simulink model "ADCSSimulator"  (R2024a)
settings: Solver=ode4  StartTime=0.0  StopTime=600  FixedStep=0.01  MaxStep=0.1  RelTol=1e-3  AbsTol=1e-3
values from neighbouring files (symbols this model uses):
  ActuatorAllocationMatrix = ActuatorPhysicalMatrix' * inv(ActuatorPhysicalMatrix * ActuatorPhysicalMatrix')    [set_Init.m]
  ActuatorPhysicalMatrix = [1, 0, 0, 0 ... (first row only)    [set_Init.m]
  albedo_irradiance = 300    [set_Init.m]
  b = 0    [set_Init.m]
  Cd = 2.2    [set_Init.m]
  h_bias = [0; 0; 0]    [set_Init.m]
  J = 4.0e-3 / 628    (= 6.36942675159e-06)    [set_Init.m]
  k_Bdot = ((4 * pi * 0.5236 * 0.0055) / (5677.2 * (4.5e-5)^2))    (= 3147.8423197)    [set_Init.m]
  K_E = K_T    (= 0.0022)    [set_Init.m]
  K_T = 0.0022    [set_Init.m]
  P0 = blkdiag(P0_att, P0_bias)    [set_Init.m]
  P0_att = eye(3) * initial_variance_rad2    [set_Init.m]
  PowerVoltageBus_01 = 3.3    [set_Init.m]
  PowerVoltageBus_02 = 3.3    [set_Init.m]
  PowerVoltageBus_03 = 3.3    [set_Init.m]
  PowerVoltageBus_04 = 3.3    [set_Init.m]
  PowerVoltageBus_05 = 3.3    [set_Init.m]
  PowerVoltageBus_06 = 3.3    [set_Init.m]
  PowerVoltageBus_07 = 3.3    [set_Init.m]
  PowerVoltageBus_08 = 3.3    [set_Init.m]
  PowerVoltageBus_09 = 3.3    [set_Init.m]
  PowerVoltageBus_10 = 3.3    [set_Init.m]
  PowerVoltageBus_11 = 3.3    [set_Init.m]
  PowerVoltageBus_12 = 0.0    (= 0)    [set_Init.m]
  PowerVoltageBus_13 = 0.0    (= 0)    [set_Init.m]
  PowerVoltageBus_14 = 0.0    (= 0)    [set_Init.m]
  PowerVoltageBus_15 = 0.0    (= 0)    [set_Init.m]
  R = 2.0    (= 2)    [set_Init.m]
  ressidual_m = [3e-4; -2e-4; 1e-4]    [set_Init.m]
  solar_irradiance = 1361    [set_Init.m]
  surface_areas = [A_xy, A_yz, A_xz, A_xy, A_yz, A_xz]    [set_Init.m]
  surface_normals_body = [eye(3) -eye(3)]    [set_Init.m]
  surface_positions_body = [       hx,   0,   0 ... (first row only)    [set_Init.m]
  surface_reflectivities = [0.9 0.8 0.9 0.9 0.9 0.9]    [set_Init.m]
  Switch_01 = 1    [set_Init.m]
  Switch_02 = 1    [set_Init.m]
  Switch_03 = 1    [set_Init.m]
  Switch_04 = 1    [set_Init.m]
  Switch_05 = 1    [set_Init.m]
  Switch_06 = 1    [set_Init.m]
  Switch_07 = 1    [set_Init.m]
  Switch_08 = 1    [set_Init.m]
  Switch_09 = 1    [set_Init.m]
  Switch_10 = 1    [set_Init.m]
  Switch_11 = 1    [set_Init.m]
  Switch_12 = 0    [set_Init.m]
  Switch_13 = 0    [set_Init.m]
  Switch_14 = 0    [set_Init.m]
  Switch_15 = 0    [set_Init.m]
  visSampleTime = 0.1    [set_Init.m]
undefined symbols (not defined in the file or in its folder): attitude, Controller, epoch, IAU, juliandate, Kd, km, Kp, m, rad, s, satellite, SGP4_parameters, simulator, UKF_parameters, WMM2020
libraries: sharedtransform x27, aerolibutil x22, aerolibconvert2 x18, simulink_extras x16, matrix_library x6, aerolibtransform2 x4, vrlib x2, aerolibgravity2 x2, aerolibobsolete x1, aerolibattitudesys x1, simulink x1
(part 2 of 8)

== system ADCSSimulator/ADCS/ADCS Software/Onboard Models ==
  Onboard Calendar : Inport
  Satellite Ephemeris [ICRF] : Inport  Port=2
  Transformers : Inport  Port=3
  Bus Creator : BusCreator  Inputs=2
  Bus Selector : BusSelector  OutputSignals=Satellite Position [ICRF] (m)
  Calendar1 : InportShadow
  Onboard Sun Ephemeris Calculator : Subsystem
  WMM : Subsystem
  Onboard Models : Outport
  wires:
  Calendar1/1 -> WMM/2(Calendar)
  WMM/1(Onboard Magnetic Field (T)) -> Bus Creator/2  "Onboard Magnetic Field"
  Onboard Sun Ephemeris Calculator/1(Onboard Sun Ephemeris [ICRF]) -> Bus Creator/1  "Onboard Sun Ephemeris"
  Transformers/1 -> WMM/3(Transformers)
  Satellite Ephemeris [ICRF]/1 -> Bus Selector/1
  Onboard Calendar/1 -> Onboard Sun Ephemeris Calculator/1(Onboard Calendar)
  Bus Selector/1 -> WMM/1(Satellite Position [ICRF] (m))  "<Satellite Position [ICRF] (m)>"
  Bus Creator/1 -> Onboard Models/1

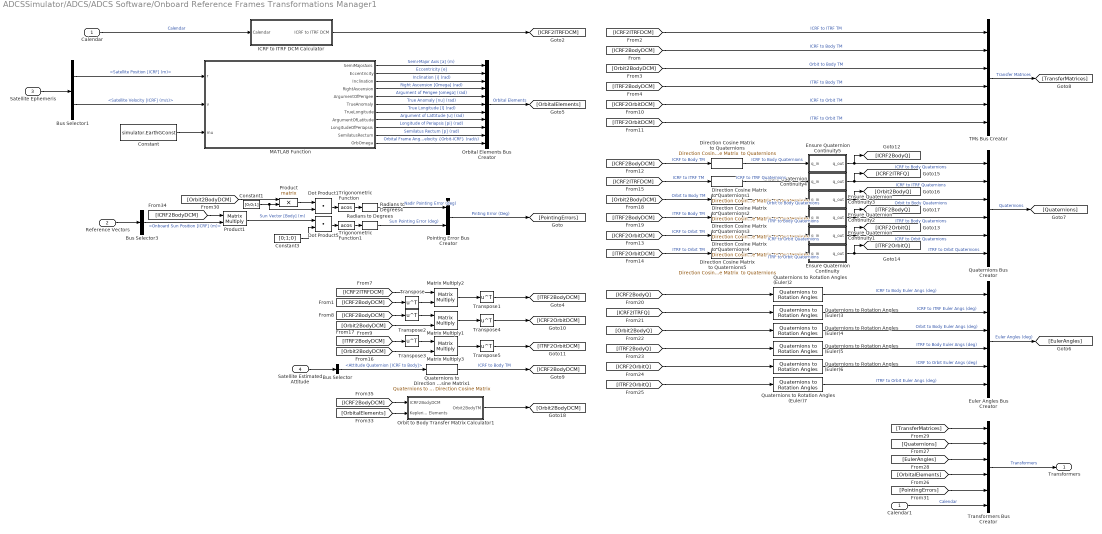
== system ADCSSimulator/ADCS/ADCS Software/Onboard Reference Frames Transformations Manager1 ==
  Calendar : Inport
  Reference Vectors : Inport  Port=2
  Satellite Ephemeris : Inport  Port=3
  Satellite Estimated Attitude : Inport  Port=4
  Bus Selector : BusSelector  OutputSignals=Attitude Quaternion [ICRF to Body]
  Bus Selector1 : BusSelector  OutputSignals=Satellite Position [ICRF] (m),Satellite Velocity [ICRF] (m/s)
  Bus Selector3 : BusSelector  OutputSignals=Onboard Sun Ephemeris.Onboard Sun Position [ICRF] (m)
  Calendar1 : InportShadow
  Constant : Constant  Value=simulator.EarthGConst
  Constant1 : Constant  Value=[0;0;1]
  Constant3 : Constant  Value=[0;1;0]
  Direction Cosine Matrix to Quaternions{,1..5} (6 alike) : sharedtransform/Direction Cosine Matrix  to Quaternions  aMode=0  action=None  tolerance=eps(2)
  Dot Product1 : DotProduct  OutDataTypeStr=Inherit: Inherit via internal rule
  Dot Product5 : DotProduct  OutDataTypeStr=Inherit: Inherit via internal rule
  Ensure Quaternion Continuity : Subsystem
  Ensure Quaternion Continuity1 : Subsystem
  Ensure Quaternion Continuity2 : Subsystem
  Ensure Quaternion Continuity3 : Subsystem
  Ensure Quaternion Continuity4 : Subsystem
  Ensure Quaternion Continuity5 : Subsystem
  Euler Angles Bus Creator : BusCreator  Inputs=6
  ICRF to ITRF DCM Calculator : Subsystem
  MATLAB Function : MATLAB Function  TreatAsAtomicUnit=on
  Matrix Multiply1 : Product  Multiplication=Matrix(*)
  Matrix Multiply2 : Product  Multiplication=Matrix(*)
  Matrix Multiply3 : Product  Multiplication=Matrix(*)
  Orbit to Body Transfer Matrix Calculator1 : Subsystem
  Orbital Elements Bus Creator : BusCreator  Inputs=11
  Pointing Error Bus Creator : BusCreator  Inputs=2
  Product : Product  Multiplication=Matrix(*)
  Product1 : Product  Multiplication=Matrix(*)
  Quaternions Bus Creator : BusCreator  Inputs=6
  Quaternions to Direction Cosine Matrix1 : sharedtransform/Quaternions to  Direction Cosine Matrix  aMode=aMode
  Quaternions to Rotation Angles (Euler){2..7} (6 alike) : sharedtransform/Quaternions to Rotation Angles  rotationOrder=XYZ  aMode=aMode
  Radians to Degrees : simulink_extras/Transformations/Radians to Degrees
  Radians to Degrees4 : simulink_extras/Transformations/Radians to Degrees
  TMs Bus Creator : BusCreator  Inputs=6
  Transformers Bus Creator : BusCreator  Inputs=6
  Transpose{,1..5} (6 alike) : Math  Operator=transpose
  Trigonometric Function : Trigonometry  Operator=acos
  Trigonometric Function1 : Trigonometry  Operator=acos  OutputSignalType=real
  Transformers : Outport
  wires:
  MATLAB Function/7(TrueLongitude) -> Orbital Elements Bus Creator/7  "True Longitude [l] (rad)"
  Ensure Quaternion Continuity3/1(q_out) -> Quaternions Bus Creator/3, [Orbit2BodyQ]  "Orbit to Body Quaternions"
  [Orbit2BodyQ] -> Quaternions to Rotation Angles (Euler)4/1
  [ITRF2OrbitQ] -> Quaternions to Rotation Angles (Euler)7/1
  [ITRF2OrbitDCM] -> Direction Cosine Matrix to Quaternions5/1  "ITRF to Orbit TM"
  Bus Selector1/2 -> MATLAB Function/2(v)  "<Satellite Velocity [ICRF] (m/s)>"
  [ICRF2ITRFQ] -> Quaternions to Rotation Angles (Euler)3/1
  [ICRF2OrbitQ] -> Quaternions to Rotation Angles (Euler)6/1
  [ICRF2BodyDCM] -> Transpose2/1
  [EulerAngles] -> Transformers Bus Creator/3
  MATLAB Function/6(TrueAnomaly) -> Orbital Elements Bus Creator/6  "True Anomaly [nu] (rad)"
  MATLAB Function/5(ArgumentOfPerigee) -> Orbital Elements Bus Creator/5  "Argument of Perigee [omega] (rad)"
  Transformers Bus Creator/1 -> Transformers/1  "Transformers"
  MATLAB Function/4(RightAscension) -> Orbital Elements Bus Creator/4  "Right Ascension [Omega] (rad)"
  MATLAB Function/10(SemilatusRectum) -> Orbital Elements Bus Creator/10  "Semilatus Rectum [p] (rad)"
  MATLAB Function/9(LongitudeOfPeriapsis) -> Orbital Elements Bus Creator/9  "Longitude of Periapsis [pi] (rad)"
  Ensure Quaternion Continuity1/1(q_out) -> Quaternions Bus Creator/5, [ICRF2OrbitQ]  "ICRF to Orbit Quaternions"
  MATLAB Function/8(ArgumentOfLatitude) -> Orbital Elements Bus Creator/8  "Argument of Lattitude [u] (rad)"
  MATLAB Function/1(SemiMajorAxis) -> Orbital Elements Bus Creator/1  "Semi-Major Axis [a] (m)"
  Reference Vectors/1 -> Bus Selector3/1
  Dot Product5/1 -> Trigonometric Function1/1
  [ICRF2BodyDCM] -> Transpose/1
  Matrix Multiply2/1 -> Transpose1/1
  Bus Selector1/1 -> MATLAB Function/1(r)  "<Satellite Position [ICRF] (m)>"
  [Orbit2BodyDCM] -> Matrix Multiply1/2
  Orbital Elements Bus Creator/1 -> [OrbitalElements]  "Orbital Elements"
  Transpose1/1 -> [ITRF2BodyDCM]
  Trigonometric Function/1 -> Radians to Degrees4/1
  Matrix Multiply3/1 -> Transpose5/1
  Constant3/1 -> Dot Product5/2
  [OrbitalElements] -> Transformers Bus Creator/4
  [ITRF2BodyDCM] -> Transpose3/1
  [Orbit2BodyDCM] -> Matrix Multiply3/2
  Radians to Degrees4/1 -> Pointing Error Bus Creator/1  "Nadir Pointing Error (deg)"
  Radians to Degrees/1 -> Pointing Error Bus Creator/2  "Sun Pointing Error (deg)"
  Calendar/1 -> ICRF to ITRF DCM Calculator/1(Calendar)  "Calendar"
  Pointing Error Bus Creator/1 -> [PointingErrors]  "Pinting Error (Deg)"
  MATLAB Function/11(OrbOmega) -> Orbital Elements Bus Creator/11  "Orbital Frame Angular Velocity {Orbit-ICRF} (rad/s)"
  Constant/1 -> MATLAB Function/3(mu)
  [Orbit2BodyDCM] -> Direction Cosine Matrix to Quaternions2/1  "Orbit to Body TM"
  [ICRF2ITRFDCM] -> TMs Bus Creator/1  "ICRF to ITRF TM"
  [ICRF2BodyDCM] -> TMs Bus Creator/2  "ICRF to Body TM"
  [PointingErrors] -> Transformers Bus Creator/5
  Transpose/1 -> Matrix Multiply2/2
  [Orbit2BodyDCM] -> Product/1
  Direction Cosine Matrix to Quaternions/1 -> Ensure Quaternion Continuity5/1(q_in)  "ICRF to Body Quaternions"
  [ICRF2OrbitDCM] -> TMs Bus Creator/5  "ICRF to Orbit TM"
  Ensure Quaternion Continuity/1(q_out) -> Quaternions Bus Creator/6, [ITRF2OrbitQ]  "ITRF to Orbit Quaternions"
  Direction Cosine Matrix to Quaternions3/1 -> Ensure Quaternion Continuity2/1(q_in)  "ITRF to Body Quaternions"
  [ICRF2BodyQ] -> Quaternions to Rotation Angles (Euler)2/1
  Constant1/1 -> Product/2, Dot Product1/2
  [ITRF2BodyDCM] -> TMs Bus Creator/4  "ITRF to Body TM"
  Quaternions to Rotation Angles (Euler)7/1 -> Euler Angles Bus Creator/6  "ITRF to Orbit Euler Angs (deg)"
  [Quaternions] -> Transformers Bus Creator/2
  [ITRF2OrbitDCM] -> TMs Bus Creator/6  "ITRF to Orbit TM"
  [ICRF2ITRFDCM] -> Matrix Multiply2/1
  Bus Selector/1 -> Quaternions to Direction Cosine Matrix1/1  "<Attitude Quaternion [ICRF to Body]>"
  Calendar1/1 -> Transformers Bus Creator/6  "Calendar"
  MATLAB Function/2(Eccentricity) -> Orbital Elements Bus Creator/2  "Eccentricity [e]"
  Ensure Quaternion Continuity4/1(q_out) -> Quaternions Bus Creator/2, [ICRF2ITRFQ]  "ICRF to ITRF Quaternions"
  Satellite Ephemeris/1 -> Bus Selector1/1
  Quaternions Bus Creator/1 -> [Quaternions]  "Quaternions"
  [ICRF2ITRFDCM] -> Direction Cosine Matrix to Quaternions1/1  "ICRF to ITRF TM"
  Matrix Multiply1/1 -> Transpose4/1
  Direction Cosine Matrix to Quaternions5/1 -> Ensure Quaternion Continuity/1(q_in)  "ITRF to Orbit Quaternions"
  Direction Cosine Matrix to Quaternions4/1 -> Ensure Quaternion Continuity1/1(q_in)  "ICRF to Orbit Quaternions"
  TMs Bus Creator/1 -> [TransferMatrices]  "Transfer Matrices"
  [ITRF2BodyDCM] -> Direction Cosine Matrix to Quaternions3/1  "ITRF to Body TM"
  Product1/1 -> Dot Product5/1  "Sun Vector [Body] (m)"
  Product/1 -> Dot Product1/1
  Ensure Quaternion Continuity2/1(q_out) -> Quaternions Bus Creator/4, [ITRF2BodyQ]  "ITRF to Body Quaternions"
  Direction Cosine Matrix to Quaternions2/1 -> Ensure Quaternion Continuity3/1(q_in)  "Orbit to Body Quaternions"
  Ensure Quaternion Continuity5/1(q_out) -> Quaternions Bus Creator/1, [ICRF2BodyQ]  "ICRF to Body Quaternions"
  Quaternions to Rotation Angles (Euler)5/1 -> Euler Angles Bus Creator/4  "ITRF to Body Euler Angs (deg)"
  Dot Product1/1 -> Trigonometric Function/1
  Direction Cosine Matrix to Quaternions1/1 -> Ensure Quaternion Continuity4/1(q_in)  "ICRF to ITRF Quaternions"
  Quaternions to Rotation Angles (Euler)2/1 -> Euler Angles Bus Creator/1  "ICRF to Body Euler Angs (deg)"
  Quaternions to Rotation Angles (Euler)3/1 -> Euler Angles Bus Creator/2  "ICRF to ITRF Euler Angs (deg)"
  Euler Angles Bus Creator/1 -> [EulerAngles]  "Euler Angles (deg)"
  MATLAB Function/3(Inclination) -> Orbital Elements Bus Creator/3  "Inclination [i] (rad)"
  [TransferMatrices] -> Transformers Bus Creator/1
  [ICRF2OrbitDCM] -> Direction Cosine Matrix to Quaternions4/1  "ICRF to Orbit TM"
  Quaternions to Rotation Angles (Euler)6/1 -> Euler Angles Bus Creator/5  "ICRF to Orbit Euler Angs (deg)"
  [ITRF2BodyQ] -> Quaternions to Rotation Angles (Euler)5/1
  [Orbit2BodyDCM] -> TMs Bus Creator/3  "Orbit to Body TM"
  Trigonometric Function1/1 -> Radians to Degrees/1
  Quaternions to Rotation Angles (Euler)4/1 -> Euler Angles Bus Creator/3  "Orbit to Body Euler Angs (deg)"
  [ICRF2BodyDCM] -> Direction Cosine Matrix to Quaternions/1  "ICRF to Body TM"
  [ICRF2BodyDCM] -> Product1/1
  Bus Selector3/1 -> Product1/2  "<Onboard Sun Position [ICRF] (m)>"
  ICRF to ITRF DCM Calculator/1(ICRF to ITRF DCM) -> [ICRF2ITRFDCM]
  Transpose2/1 -> Matrix Multiply1/1
  Transpose4/1 -> [ICRF2OrbitDCM]
  Transpose3/1 -> Matrix Multiply3/1
  Transpose5/1 -> [ITRF2OrbitDCM]
  [OrbitalElements] -> Orbit to Body Transfer Matrix Calculator1/2(Keplerian Elements)
  [ICRF2BodyDCM] -> Orbit to Body Transfer Matrix Calculator1/1(ICRF2BodyDCM)
  Quaternions to Direction Cosine Matrix1/1 -> [ICRF2BodyDCM]  "ICRF to Body TM"
  Orbit to Body Transfer Matrix Calculator1/1(Orbit2BodyTM) -> [Orbit2BodyDCM]
  Satellite Estimated Attitude/1 -> Bus Selector/1

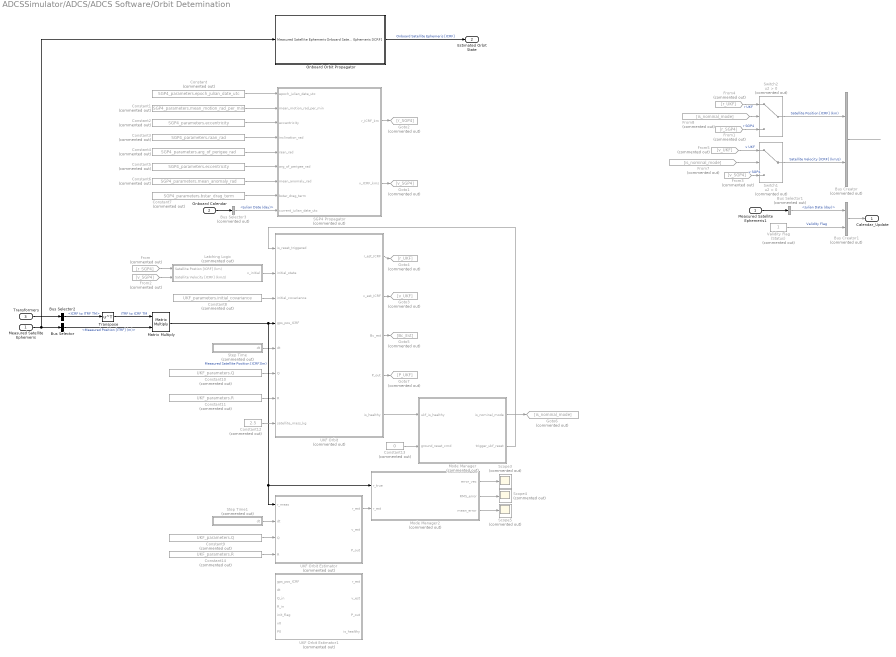
== system ADCSSimulator/ADCS/ADCS Software/Orbit Detemination ==
  Measured Satellite Ephemeris : Inport
  Onboard Calendar : Inport  Port=2
  Transformers : Inport  Port=3
  Bus Creator : BusCreator  Commented=on  Inputs=2
  Bus Creator1 : BusCreator  Commented=on  Inputs=2
  Bus Selector : BusSelector  OutputSignals=Measured Position [ITRF] (m)
  Bus Selector1 : BusSelector  Commented=on  OutputSignals=Julian Date (day)
  Bus Selector2 : BusSelector  OutputSignals=Transfer Matrices.ICRF to ITRF TM
  Bus Selector3 : BusSelector  Commented=on  OutputSignals=Julian Date (day)
  Constant : Constant  Commented=on  Value=SGP4_parameters.epoch_julian_date_utc
  Constant1 : Constant  Commented=on  Value=SGP4_parameters.mean_motion_rad_per_min
  Constant10 : Constant  Commented=on  Value=UKF_parameters.Q
  Constant11 : Constant  Commented=on  Value=UKF_parameters.R
  Constant12 : Constant  Commented=on  Value=2.5
  Constant13 : Constant  Commented=on  Value=0
  Constant14 : Constant  Commented=on  Value=UKF_parameters.R
  Constant2 : Constant  Commented=on  Value=SGP4_parameters.eccentricity
  Constant3 : Constant  Commented=on  Value=SGP4_parameters.raan_rad
  Constant4 : Constant  Commented=on  Value=SGP4_parameters.arg_of_perigee_rad
  Constant5 : Constant  Commented=on  Value=SGP4_parameters.eccentricity
  Constant6 : Constant  Commented=on  Value=SGP4_parameters.mean_anomaly_rad
  Constant7 : Constant  Commented=on  Value=SGP4_parameters.bstar_drag_term
  Constant8 : Constant  Commented=on  Value=UKF_parameters.initial_covariance
  Constant9 : Constant  Commented=on  Value=UKF_parameters.Q
  From : From  Commented=on  GotoTag=r_SGP4
  From1 : From  Commented=on  GotoTag=r_SGP4
  From2 : From  Commented=on  GotoTag=v_SGP4
  From3 : From  Commented=on  GotoTag=v_SGP4
  From4 : From  Commented=on  GotoTag=r_UKF
  From5 : From  Commented=on  GotoTag=v_UKF
  From7 : From  Commented=on  GotoTag=is_nominal_mode
  From8 : From  Commented=on  GotoTag=is_nominal_mode
  Goto1 : Goto  Commented=on  GotoTag=v_SGP4
  Goto2 : Goto  Commented=on  GotoTag=r_SGP4
  Goto3 : Goto  Commented=on  GotoTag=v_UKF
  Goto4 : Goto  Commented=on  GotoTag=r_UKF
  Goto5 : Goto  Commented=on  GotoTag=Bc_Est
  Goto6 : Goto  Commented=on  GotoTag=is_nominal_mode
  Goto7 : Goto  Commented=on  GotoTag=P_UKF
  Latching Logic : Subsystem  Commented=on
  Matrix Multiply : Product  Multiplication=Matrix(*)
  Measured Satellite Ephemeris1 : InportShadow
  Mode Manager : MATLAB Function  Commented=on  TreatAsAtomicUnit=on
  Mode Manager2 : MATLAB Function  Commented=on  TreatAsAtomicUnit=on
  "Onboard Orbit Propagator " : Subsystem
  SGP4 Propagator : MATLAB Function  Commented=on  TreatAsAtomicUnit=on
  Scope3 : Scope  Commented=on
  Scope4 : Scope  Commented=on
  Scope5 : Scope  Commented=on
  Step Time : Subsystem  Commented=on
  Step Time1 : Subsystem  Commented=on
  Switch1 : Switch  Commented=on  Criteria=u2 > Threshold  SaturateOnIntegerOverflow=off  InputSameDT=off
  Switch2 : Switch  Commented=on  Criteria=u2 > Threshold  SaturateOnIntegerOverflow=off  InputSameDT=off
  Transpose : Math  Operator=transpose
  "UKF Orbit " : MATLAB Function  Commented=on  TreatAsAtomicUnit=on  SystemSampleTime=1
  UKF Orbit Estimator : MATLAB Function  Commented=on  TreatAsAtomicUnit=on
  UKF Orbit Estimator1 : MATLAB Function  Commented=on  TreatAsAtomicUnit=on
  Validity Flag (Status) : Constant  Commented=on
  Calendar_Update : Outport
  Estimated Orbit State : Outport  Port=2
  wires:
  Constant/1 -> SGP4 Propagator/1(epoch_julian_date_utc)
  Constant1/1 -> SGP4 Propagator/2(mean_motion_rad_per_min)
  Constant2/1 -> SGP4 Propagator/3(eccentricity)
  Constant4/1 -> SGP4 Propagator/5(raan_rad)
  Constant5/1 -> SGP4 Propagator/6(arg_of_perigee_rad)
  Constant3/1 -> SGP4 Propagator/4(inclination_rad)
  Bus Selector/1 -> Matrix Multiply/2  "<Measured Position [ITRF] (m)>"
  Step Time/1(dt) -> "UKF Orbit "/5(dt)
  Constant8/1 -> "UKF Orbit "/3(initial_covariance)
  Constant10/1 -> "UKF Orbit "/6(Q)
  Constant11/1 -> "UKF Orbit "/7(R)
  Latching Logic/1(x_initial) -> "UKF Orbit "/2(initial_state)
  SGP4 Propagator/2(v_ICRF_kms) -> Goto1/1
  SGP4 Propagator/1(r_ICRF_km) -> Goto2/1
  From/1 -> Latching Logic/1(Satellite Postion [ICRF] (km))
  From2/1 -> Latching Logic/2(Satellite Velocity [ICRF] (km/s))
  "UKF Orbit "/3(Bc_est) -> Goto5/1
  Bus Creator/1 -> ?
  "UKF Orbit "/2(v_est_ICRF) -> Goto3/1
  "UKF Orbit "/1(r_est_ICRF) -> Goto4/1
  Switch2/1 -> Bus Creator/1  "Satellite Position [ICRF] (km)"
  Switch1/1 -> Bus Creator/2  "Satellite Velocity [ICRF] (km/s)"
  Constant6/1 -> SGP4 Propagator/7(mean_anomaly_rad)
  Measured Satellite Ephemeris1/1 -> Bus Selector1/1
  Bus Selector1/1 -> Bus Creator1/1  "<Julian Date (day)>"
  Validity Flag (Status)/1 -> Bus Creator1/2  "Validity Flag"
  Bus Creator1/1 -> Calendar_Update/1
  Bus Selector2/1 -> Transpose/1  "<ICRF to ITRF TM>"
  Transformers/1 -> Bus Selector2/1
  Transpose/1 -> Matrix Multiply/1  "ITRF to ICRF TM"
  Matrix Multiply/1 -> "UKF Orbit "/4(gps_pos_ICRF), UKF Orbit Estimator/1(r_meas), Mode Manager2/1(r_true)  "Measured Satellite Position [ICRF](m)"
  Onboard Calendar/1 -> Bus Selector3/1
  Bus Selector3/1 -> SGP4 Propagator/9(current_julian_date_utc)  "<Julian Date (day)>"
  Constant12/1 -> "UKF Orbit "/8(satellite_mass_kg)
  Mode Manager/2(trigger_ukf_reset) -> "UKF Orbit "/1(is_reset_triggered)
  "UKF Orbit "/5(is_healthy) -> Mode Manager/1(ukf_is_healthy)
  From1/1 -> Switch2/3  "r SGP4"
  From4/1 -> Switch2/1  "r UKF"
  Constant13/1 -> Mode Manager/2(ground_reset_cmd)
  Mode Manager/1(is_nominal_mode) -> Goto6/1
  From8/1 -> Switch2/2
  From7/1 -> Switch1/2
  From3/1 -> Switch1/3  "v SGP4"
  From5/1 -> Switch1/1  "v UKF"
  "UKF Orbit "/4(P_out) -> Goto7/1
  Constant7/1 -> SGP4 Propagator/8(bstar_drag_term)
  "Onboard Orbit Propagator "/1(Onboard Satellite Ephemeris [ICRF]) -> Estimated Orbit State/1  "Onboard Satellite Ephemeris [ICRF]"
  Measured Satellite Ephemeris/1 -> "Onboard Orbit Propagator "/1(Measured Satellite Ephemeris), Bus Selector/1
  Constant14/1 -> UKF Orbit Estimator/4(R)
  Step Time1/1(dt) -> UKF Orbit Estimator/2(dt)
  Constant9/1 -> UKF Orbit Estimator/3(Q)
  UKF Orbit Estimator/1(r_est) -> Mode Manager2/2(r_est)
  Mode Manager2/1(error_vec) -> Scope3/1
  Mode Manager2/2(RMS_error) -> Scope4/1
  Mode Manager2/3(mean_error) -> Scope5/1

== system ADCSSimulator/ADCS/Environment Model/Attitude Dynamics & Kynematics ==
  Transformers : Inport
  Actuators : Inport  Port=2
  Disturbances : Inport  Port=3
  Bus Selector : BusSelector  OutputSignals=Transfer Matrices.Orbit to Body TM,Orbital Elements.Orbital Frame Angular Velocity {Orbit-ICRF} (rad/s)
  Bus Selector1 : BusSelector  OutputSignals=RWs.RWs Torque [Body](Nm)
  Bus Selector2 : BusSelector  OutputSignals=MTQs.MTQs Torque [Body] (Nm)
  Constant : Constant  Value=satellite.MOI
  Constant2 : Constant  Value=satellite.InvMOI
  Constant3 : Constant  Value=[attitude.P0; attitude.Q0; attitude.R0]
  Constant4 : Constant  Value=[attitude.Phi0; attitude.Theta0; attitude.Psi0]
  Cross Product : matrix_library/Cross Product
  Gain : Gain  Gain=0.5
  Gain1 : Gain
  Integrator : Integrator  InitialConditionSource=external  IgnoreLimit=on  ContinuousStateAttributes={'P','Q','R'}
  Integrator1 : Integrator  InitialConditionSource=external  ContinuousStateAttributes={'q0','q1','q2','q3'}
  Interpreted MATLAB Function : MATLABFcn  MATLABFcn=[0,-u(1),-u(2),-u(3);u(1),0,u(3),-u(2);u(2),-u(3),0,u(1);u(3),u(2),-u(1),0]  OutputDimensions=[4,4]  OutputSignalType=real  Output1D=off
  Product : Product  Inputs=*/
  Product{1..4} (4 alike) : Product  Multiplication=Matrix(*)
  Rotation Angles to Quaternions : sharedtransform/Rotation Angles to Quaternions  rotationOrder=XYZ  aMode=aMode
  Satellite Attitude Bus Creator : BusCreator  Inputs=3
  Sum : Sum  Inputs=|+-
  Sum1 : Sum  Inputs=+++
  Sum3 : Sum  Inputs=|-+
  sqrt : Subsystem
  Satellite Attitude : Outport
  wires:
  Integrator/1 -> Product2/2, Cross Product/1, Satellite Attitude Bus Creator/2, Sum3/2  "Angular Velocity {Body-ICRF}(rad/s)"
  Bus Selector/2 -> Product3/2  "<Orbital Frame Angular Velocity {Orbit-ICRF} (rad/s)>"
  Constant2/1 -> Product1/1
  Interpreted MATLAB Function/1 -> Product4/1
  Satellite Attitude Bus Creator/1 -> Satellite Attitude/1  "Satellite Attitude"
  Product3/1 -> Sum3/1  "Body Frame Angular Velocity {Body-ICRF}"
  Sum1/1 -> Sum/1  "M"
  Constant4/1 -> Rotation Angles to Quaternions/1
  Transformers/1 -> Bus Selector/1
  Product1/1 -> Integrator/1  "Angular Velocity Time Rate {Body-ICRF}(rad/s^2)"
  Gain/1 -> Product4/2
  Constant3/1 -> Integrator/2
  Product4/1 -> Integrator1/1
  Bus Selector/1 -> Product3/1  "<Orbit to Body TM>"
  Integrator1/1 -> sqrt/1(u), Product/1, Satellite Attitude Bus Creator/3  "Orbit to Body Quaternions"
  Sum3/1 -> Interpreted MATLAB Function/1, Satellite Attitude Bus Creator/1  "Angular Velocity {Body-Orbit}(rad/s)"
  Actuators/1 -> Bus Selector2/1, Bus Selector1/1
  Rotation Angles to Quaternions/1 -> Integrator1/2
  Product/1 -> Gain/1
  Disturbances/1 -> Gain1/1  "Total Disturbance Torques [Body] (N.m)"
  sqrt/1(sqrt(u)) -> Product/2
  Constant/1 -> Product2/1
  Product2/1 -> Cross Product/2  "Iw"
  Cross Product/1 -> Sum/2  "w*Iw"
  Sum/1 -> Product1/2  "M-w*(Iw)"
  Bus Selector2/1 -> Sum1/1  "<MTQs Torque [Body] (Nm)>"
  Bus Selector1/1 -> Sum1/2  "<RWs Torque [Body](Nm)>"
  Gain1/1 -> Sum1/3

== system ADCSSimulator/ADCS/Environment Model/Calendar  ==
  Since Epoch (sec) : Inport  OutDataTypeStr=double  Unit=s  PortDimensions=1
  Calendar Bus Creator : BusCreator  Inputs=4
  Constant6 : Constant  Value=epoch.DecimalYear
  JD : Subsystem
  MJD : Subsystem
  Calendar : Outport
  wires:
  Since Epoch (sec)/1 -> MJD/1(Since Epoch (sec)), JD/1(Since Epoch (sec)), Calendar Bus Creator/4  "Since Epoch (sec)"
  Constant6/1 -> Calendar Bus Creator/3  "Decimal Year (year)"
  JD/1(Julian Date (day)) -> Calendar Bus Creator/1  "Julian Date (day)"
  Calendar Bus Creator/1 -> Calendar/1  "Calendar_out"
  MJD/1(Modified Julian Date (day)) -> Calendar Bus Creator/2  "Modified Julian Date (day)"

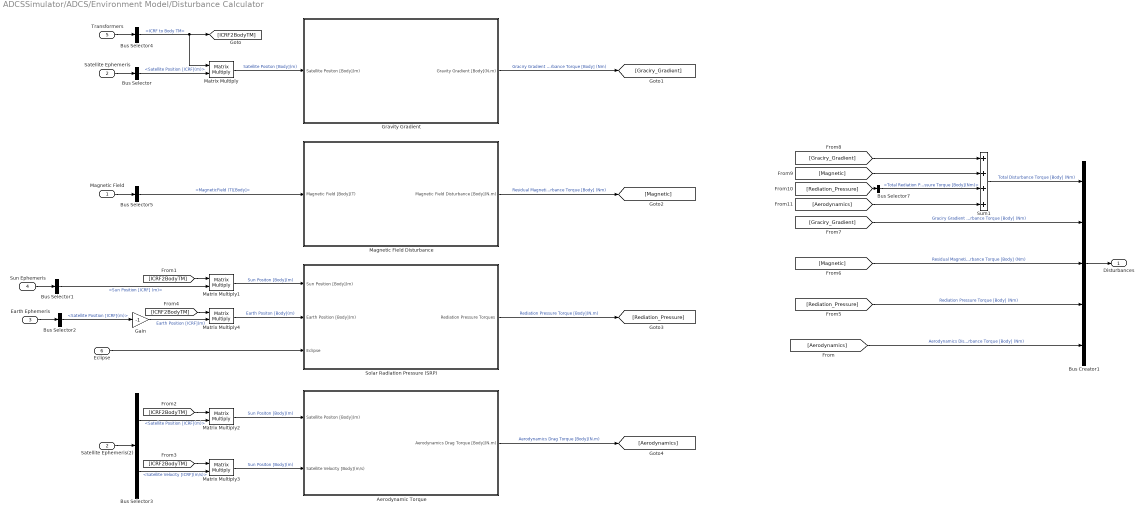
== system ADCSSimulator/ADCS/Environment Model/Disturbance Calculator ==
  Magnetic Field : Inport
  Satellite Ephemeris : Inport  Port=2
  Earth Ephemeris : Inport  Port=3
  Sun Ephemeris : Inport  Port=4
  Transformers : Inport  Port=5
  Eclipse : Inport  Port=6
  Aerodynamic Torque : Subsystem
  Bus Creator1 : BusCreator  Inputs=5
  Bus Selector : BusSelector  OutputSignals=Satellite Position [ICRF](m)
  Bus Selector1 : BusSelector  OutputSignals=Sun Position [ICRF] (m)
  Bus Selector2 : BusSelector  OutputSignals=Satellite Ephemeris [ICRF].Satellite Position [ICRF](m)
  Bus Selector3 : BusSelector  OutputSignals=Satellite Position [ICRF](m),Satellite Velocity [ICRF](m/s)
  Bus Selector4 : BusSelector  OutputSignals=Transfer Matrices.ICRF to Body TM
  Bus Selector5 : BusSelector  OutputSignals=|
      | MagneticField
      | (T)[Body]
  Bus Selector7 : BusSelector  OutputSignals=Total Rediation Pressure Torque [Body](Nm)
  Gain : Gain  Gain=-1
  Gravity Gradient : Subsystem
  Magnetic Field Disturbance : Subsystem
  Matrix Multiply{,1..4} (5 alike) : Product  Multiplication=Matrix(*)
  Satellite Ephemeris(2) : InportShadow  Port=2
  Solar Radiation Pressure (SRP) : Subsystem
  Sum1 : Sum  Inputs=++++
  Disturbances : Outport
  wires:
  Solar Radiation Pressure (SRP)/1(Rediation Pressure Torques) -> [Rediation_Pressure]  "Rediation Pressure Torque [Body](N.m)"
  Aerodynamic Torque/1(Aerodynamics Drag Torque [Body](N.m)) -> [Aerodynamics]  "Aerodynamics Drag Torque [Body](N.m)"
  Magnetic Field/1 -> Bus Selector5/1
  Satellite Ephemeris/1 -> Bus Selector/1
  Satellite Ephemeris(2)/1 -> Bus Selector3/1
  Sun Ephemeris/1 -> Bus Selector1/1
  Transformers/1 -> Bus Selector4/1
  Bus Selector4/1 -> [ICRF2BodyTM], Matrix Multiply/1  "<ICRF to Body TM>"
  Bus Selector/1 -> Matrix Multiply/2  "<Satellite Position [ICRF](m)>"
  Matrix Multiply/1 -> Gravity Gradient/1(Satellite Positon [Body](m))  "Satellite Positon [Body](m)"
  Bus Selector5/1 -> Magnetic Field Disturbance/1(Magnetic Field [Body](T))  "<MagneticField (T)[Body]>"
  [ICRF2BodyTM] -> Matrix Multiply1/1
  Matrix Multiply1/1 -> Solar Radiation Pressure (SRP)/1(Sun Position [Body](m))  "Sun Positon [Body](m)"
  Bus Selector1/1 -> Matrix Multiply1/2  "<Sun Position [ICRF] (m)>"
  [ICRF2BodyTM] -> Matrix Multiply2/1
  Matrix Multiply2/1 -> Aerodynamic Torque/1(Satellite Positon [Body](m))  "Sun Positon [Body](m)"
  Bus Selector3/1 -> Matrix Multiply2/2  "<Satellite Position [ICRF](m)>"
  [ICRF2BodyTM] -> Matrix Multiply3/1
  Matrix Multiply3/1 -> Aerodynamic Torque/2(Satellite Velocity [Body](m/s))  "Sun Positon [Body](m)"
  Bus Selector3/2 -> Matrix Multiply3/2  "<Satellite Velocity [ICRF](m/s)>"
  Earth Ephemeris/1 -> Bus Selector2/1
  [ICRF2BodyTM] -> Matrix Multiply4/1
  Bus Selector2/1 -> Gain/1  "<Satellite Position [ICRF](m)>"
  Gain/1 -> Matrix Multiply4/2  "Earth Position [ICRF](m)"
  Matrix Multiply4/1 -> Solar Radiation Pressure (SRP)/2(Earth Position [Body](m))  "Earth Positon [Body](m)"
  Magnetic Field Disturbance/1(Magnetic Field Disturbance [Body](N.m)) -> [Magnetic]  "Residual Magnetic Disturbance Torque [Body] (Nm)"
  Gravity Gradient/1(Gravity Gradient [Body](N.m)) -> [Graciry_Gradient]  "Graciry Gradient Disturbance Torque [Body] (Nm)"
  [Rediation_Pressure] -> Bus Selector7/1
  [Magnetic] -> Sum1/2
  Bus Creator1/1 -> Disturbances/1
  [Magnetic] -> Bus Creator1/3  "Residual Magnetic Disturbance Torque [Body] (Nm)"
  [Graciry_Gradient] -> Sum1/1
  [Rediation_Pressure] -> Bus Creator1/4  "Rediation Pressure Torque [Body] (Nm)"
  [Aerodynamics] -> Bus Creator1/5  "Aerodynamics Disturbance Torque [Body] (Nm)"
  [Aerodynamics] -> Sum1/4
  [Graciry_Gradient] -> Bus Creator1/2  "Graciry Gradient Disturbance Torque [Body] (Nm)"
  Sum1/1 -> Bus Creator1/1  "Total Disturbance Torque [Body] (Nm)"
  Eclipse/1 -> Solar Radiation Pressure (SRP)/3(Eclipse)
  Bus Selector7/1 -> Sum1/3  "<Total Rediation Pressure Torque [Body](Nm)>"

== system ADCSSimulator/ADCS/Environment Model/IGRF [ECEF] ==
  Satellite Ephemeris [ICRF] : Inport
  Calendar : Inport  Port=2
  Transformers : Inport  Port=3
  Bus Selector : BusSelector  OutputSignals=Decimal Year (year)
  Bus Selector1 : BusSelector  OutputSignals=Transfer Matrices.ITRF to Body TM
  Bus Selector2 : BusSelector  OutputSignals=Transfer Matrices.ICRF to ITRF TM
  Bus Selector3 : BusSelector  OutputSignals=Satellite Position [ICRF](m)
  Bus Selector4 : BusSelector  OutputSignals=Transfer Matrices.ICRF to ITRF TM
  Convert to Teslla : Gain  Gain=10^-9  Multiplication=Matrix(K*u)
  Demux : Demux  Outputs=2
  Direction Cosine Matrix ECEF to NED : aerolibtransform2/Direction Cosine Matrix ECEF to NED
  Divide{,1..3} (4 alike) : Product  Inputs=**  Multiplication=Matrix(*)
  ECEF Position to LLA : ECEF2LLA
  Magnetic Field Bus Creator : BusCreator  Inputs=3
  Mux : Mux  Inputs=2
  Reshape : Reshape  OutputDimensionality=Customize  OutputDimensions=[3,1]
  Transpose : Math  Operator=transpose
  Transpose1 : Math  Operator=transpose
  World Magnetic Model : aerolibgravity2/World Magnetic Model  model=WMM2020 (2020-2025)  customFile='WMM2020.COF'  units=Metric (MKS)  time_in=on  month=January  day=1  year=2020  action=Error  h_out=off  dec_out=off  inc_out=off  ti_out=off
  Magnetic Field (T) : Outport
  wires:
  [Latitude_deg] -> World Magnetic Model/2  "Latitude (deg)"
  Transpose/1 -> Divide/1
  Demux/1 -> [Latitude_deg]
  [Altitude_m] -> World Magnetic Model/1  "Altitude (m)"
  Reshape/1 -> Divide3/2, Magnetic Field Bus Creator/2, Divide1/2  "Magnetic Field (T) [ITRF]"
  Direction Cosine Matrix ECEF to NED/1 -> Transpose/1
  Magnetic Field Bus Creator/1 -> Magnetic Field (T)/1  "Magnetic Field (T)"
  Mux/1 -> Direction Cosine Matrix ECEF to NED/1
  Transformers/1 -> Bus Selector1/1, Bus Selector2/1, Bus Selector4/1
  [Latitude_deg] -> Mux/1  "Latitude (deg)"
  [Longitude_deg] -> Mux/2  "Longitude (deg)"
  ECEF Position to LLA/2 -> [Altitude_m]
  Demux/2 -> [Longitude_deg]
  Divide/1 -> Convert to Teslla/1
  Convert to Teslla/1 -> Reshape/1
  Calendar/1 -> Bus Selector/1
  ECEF Position to LLA/1 -> Demux/1
  Divide2/1 -> ECEF Position to LLA/1  "Satellite Position [ITRF] (m)"
  [Longitude_deg] -> World Magnetic Model/3  "Longitude (deg)"
  Bus Selector/1 -> World Magnetic Model/4  "<Decimal Year (year)>"
  Divide1/1 -> Magnetic Field Bus Creator/3  "MagneticField (T)[Body]"
  World Magnetic Model/1 -> Divide/2
  Bus Selector1/1 -> Divide1/1  "<ITRF to Body TM>"
  Satellite Ephemeris [ICRF]/1 -> Bus Selector3/1  "Satellite Ephemeris [ICRF]"
  Bus Selector2/1 -> Divide2/1  "<ICRF to ITRF TM>"
  Bus Selector3/1 -> Divide2/2  "<Satellite Position [ICRF](m)>"
  Bus Selector4/1 -> Transpose1/1  "<ICRF to ITRF TM>"
  Transpose1/1 -> Divide3/1  "ITRF to ICRF TM"
  Divide3/1 -> Magnetic Field Bus Creator/1  "MagneticField (T)[ICRF]"

== system ADCSSimulator/ADCS/Environment Model/Orbit Eclipse Calculator ==
  Sun Ephemeris [ICRF] : Inport
  Satellite Ephemeris [ICRF] : Inport  Port=2
  Bus Selector : BusSelector  OutputSignals=Satellite Position [ICRF](m)
  Bus Selector1 : BusSelector  OutputSignals=Sun Position [ICRF] (m)
  MATLAB Function1 : MATLAB Function  TreatAsAtomicUnit=on
  Eclipse : Outport
  wires:
  Sun Ephemeris [ICRF]/1 -> Bus Selector1/1
  Satellite Ephemeris [ICRF]/1 -> Bus Selector/1
  Bus Selector/1 -> MATLAB Function1/1(r_sat)  "<Satellite Position [ICRF](m)>"
  MATLAB Function1/1(isInEclipse) -> Eclipse/1
  Bus Selector1/1 -> MATLAB Function1/2(r_sun)  "<Sun Position [ICRF] (m)>"

== system ADCSSimulator/ADCS/Environment Model/Orbit Propagator ==
  Bus Creator : BusCreator  Inputs=2
  Orbit Propagator Numerical (high precision) : OrbitPropagator  propagator=Numerical (high precision)  startDate=juliandate(epoch.Year, epoch.Month, epoch.Day, epoch.Hour, epoch.Minute, epoch.Second)  dateOut=off  orbitType=Circular inclined  semiMajorAxis=Semi_major_axis  inclination=Inclination  raan=RAAN  argLat=Argument_of_latitude  inertialPosition=[3649700.0 3308200.0 -4676600.0]  inertialVelocity=[-2750.8 6666.4 2573.4]  fixedPosition=[-4142689.0 -2676864.7 -4669861.6]  fixedVelocity=[1452.7 -6720.7 2568.1]  customR=3396200  customMu=4.305e13  customJ2=1.0826269e-03  customOmega=4.06125949e-3
  Satellite Ephemeris [ICRF] : Outport
  wires:
  Bus Creator/1 -> Satellite Ephemeris [ICRF]/1  "Satellite Ephemeris [ICRF]"
  Orbit Propagator Numerical (high precision)/1 -> Bus Creator/1  "Satellite Position [ICRF](m)"
  Orbit Propagator Numerical (high precision)/2 -> Bus Creator/2  "Satellite Velocity [ICRF](m/s)"

== system ADCSSimulator/ADCS/Environment Model/Planetary Ephemeris Calculator ==
  Calendar : Inport
  Bus Selector : BusSelector  OutputSignals=Julian Date (day)
  Length Conversion : aerolibconvert2/Length Conversion  IU=km  OU=m
  Length Conversion1 : aerolibconvert2/Length Conversion  IU=km  OU=m
  Moon Ephemeris Bus Creator : BusCreator  Inputs=2
  Moon Ephemeris Calculator : PlanetaryEphem
  Sun Ephemeris Bus Creator : BusCreator  Inputs=2
  Sun Ephemeris Calculator : PlanetaryEphem  target=Sun
  Velocity Conversion : aerolibconvert2/Velocity Conversion  IU=km/s  OU=m/s
  Velocity Conversion1 : aerolibconvert2/Velocity Conversion  IU=km/s  OU=m/s
  Sun Ephemeris [ICRF] : Outport
  Moon Ephemeris [ICRF] : Outport  Port=2
  wires:
  Moon Ephemeris Bus Creator/1 -> Moon Ephemeris [ICRF]/1  "Moon Ephemeris [ICRF]"
  Velocity Conversion/1 -> Moon Ephemeris Bus Creator/2  "Moon Velocity [ICRF] (m/s)"
  Bus Selector/1 -> Moon Ephemeris Calculator/1, Sun Ephemeris Calculator/1  "<Julian Date (day)>"
  Moon Ephemeris Calculator/2 -> Velocity Conversion/1
  Calendar/1 -> Bus Selector/1
  Sun Ephemeris Calculator/1 -> Length Conversion1/1
  Sun Ephemeris Calculator/2 -> Velocity Conversion1/1
  Velocity Conversion1/1 -> Sun Ephemeris Bus Creator/2  "Sun Velocity [ICRF] (m/s)"
  Length Conversion/1 -> Moon Ephemeris Bus Creator/1  "Moon Position [ICRF] (m)"
  Sun Ephemeris Bus Creator/1 -> Sun Ephemeris [ICRF]/1  "Sun Ephemeris [ICRF]"
  Length Conversion1/1 -> Sun Ephemeris Bus Creator/1  "Sun Position [ICRF] (m)"
  Moon Ephemeris Calculator/1 -> Length Conversion/1

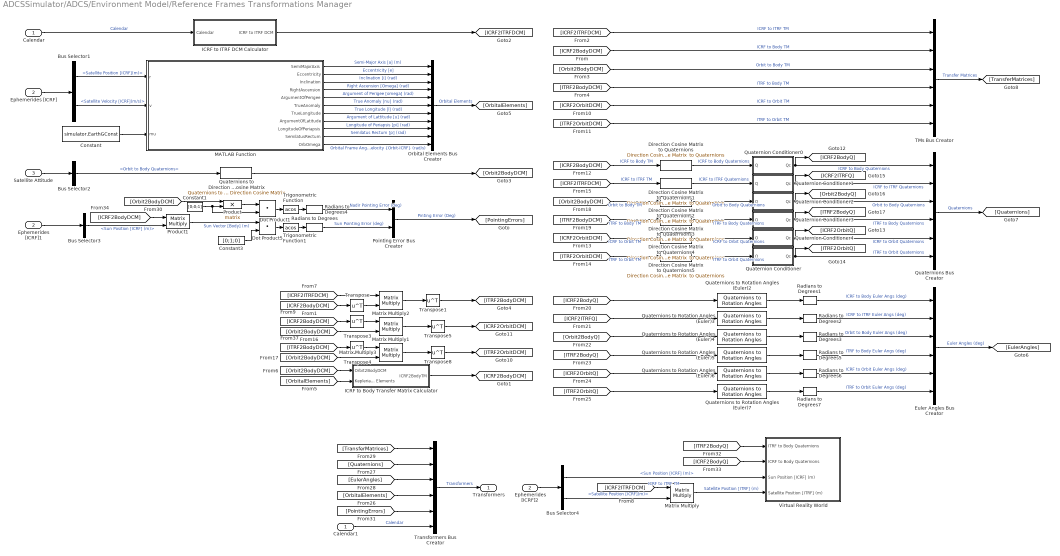
== system ADCSSimulator/ADCS/Environment Model/Reference Frames Transformations Manager ==
  Calendar : Inport
  Ephemerides [ICRF] : Inport  Port=2
  Satellite Attitude : Inport  Port=3
  Bus Selector1 : BusSelector  OutputSignals=Satellite Ephemeris [ICRF].Satellite Position [ICRF](m),Satellite Ephemeris [ICRF].Satellite Velocity [ICRF](m/s)
  Bus Selector2 : BusSelector  OutputSignals=Orbit to Body Quaternions
  Bus Selector3 : BusSelector  OutputSignals=Planetary Ephemeris [ICRF].Sun Ephemeris [ICRF].Sun Position [ICRF] (m)
  Bus Selector4 : BusSelector  OutputSignals=Planetary Ephemeris [ICRF].Sun Ephemeris [ICRF].Sun Position [ICRF] (m),Satellite Ephemeris [ICRF].Satellite Position [ICRF](m)
  Calendar1 : InportShadow
  Constant : Constant  Value=simulator.EarthGConst
  Constant1 : Constant  Value=[0;0;1]
  Constant3 : Constant  Value=[0;1;0]
  Direction Cosine Matrix to Quaternions{,1..5} (6 alike) : sharedtransform/Direction Cosine Matrix  to Quaternions  aMode=0  action=None  tolerance=eps(2)
  Dot Product1 : DotProduct  OutDataTypeStr=Inherit: Inherit via internal rule
  Dot Product5 : DotProduct  OutDataTypeStr=Inherit: Inherit via internal rule
  Ephemerides [ICRF]1 : InportShadow  Port=2
  Ephemerides [ICRF]2 : InportShadow  Port=2
  Euler Angles Bus Creator : BusCreator  Inputs=6
  ICRF to Body Transfer Matrix Calculator : Subsystem
  ICRF to ITRF DCM Calculator : Subsystem
  MATLAB Function : MATLAB Function  TreatAsAtomicUnit=on
  Matrix Multiply{,1..3} (4 alike) : Product  Multiplication=Matrix(*)
  Orbital Elements Bus Creator : BusCreator  Inputs=11
  Pointing Error Bus Creator : BusCreator  Inputs=2
  Product : Product  Multiplication=Matrix(*)
  Product1 : Product  Multiplication=Matrix(*)
  Quaternion Conditioner : Subsystem
  Quaternion Conditioner0 : Subsystem
  Quaternion Conditioner1 : Subsystem
  Quaternion Conditioner2 : Subsystem
  Quaternion Conditioner3 : Subsystem
  Quaternion Conditioner4 : Subsystem
  Quaternions Bus Creator : BusCreator  Inputs=6
  Quaternions to Direction Cosine Matrix : sharedtransform/Quaternions to  Direction Cosine Matrix  aMode=aMode
  Quaternions to Rotation Angles (Euler){2..7} (6 alike) : sharedtransform/Quaternions to Rotation Angles  rotationOrder=XYZ  aMode=aMode
  Radians to Degrees{,1..7} (8 alike) : simulink_extras/Transformations/Radians to Degrees
  TMs Bus Creator : BusCreator  Inputs=6
  Transformers Bus Creator : BusCreator  Inputs=6
  Transpose{,1,3..5,8} (6 alike) : Math  Operator=transpose
  Trigonometric Function : Trigonometry  Operator=acos
  Trigonometric Function1 : Trigonometry  Operator=acos  OutputSignalType=real
  Virtual Reality World : Subsystem  AncestorBlock=SepehrMILLib/Reference Frames Transformations Manager/Virtual Reality World  VariantControl=visSL3D
  Transformers : Outport
  wires:
  MATLAB Function/7(TrueLongitude) -> Orbital Elements Bus Creator/7  "True Longitude [l] (rad)"
  Quaternion Conditioner2/1(Qc) -> Quaternions Bus Creator/3, [Orbit2BodyQ]  "Orbit to Body Quaternions"
  [Orbit2BodyQ] -> Quaternions to Rotation Angles (Euler)4/1
  [ITRF2OrbitQ] -> Quaternions to Rotation Angles (Euler)7/1
  [ITRF2OrbitDCM] -> Direction Cosine Matrix to Quaternions5/1  "ITRF to Orbit TM"
  Bus Selector1/2 -> MATLAB Function/2(v)  "<Satellite Velocity [ICRF](m/s)>"
  [ICRF2ITRFQ] -> Quaternions to Rotation Angles (Euler)3/1
  [ICRF2OrbitQ] -> Quaternions to Rotation Angles (Euler)6/1
  [EulerAngles] -> Transformers Bus Creator/3
  MATLAB Function/6(TrueAnomaly) -> Orbital Elements Bus Creator/6  "True Anomaly [nu] (rad)"
  MATLAB Function/5(ArgumentOfPerigee) -> Orbital Elements Bus Creator/5  "Argument of Perigee [omega] (rad)"
  Bus Selector4/1 -> Virtual Reality World/3(Sun Position [ICRF] (m))  "<Sun Position [ICRF] (m)>"
  Transformers Bus Creator/1 -> Transformers/1  "Transformers"
  MATLAB Function/4(RightAscension) -> Orbital Elements Bus Creator/4  "Right Ascension [Omega] (rad)"
  MATLAB Function/10(SemilatusRectum) -> Orbital Elements Bus Creator/10  "Semilatus Rectum [p] (rad)"
  MATLAB Function/9(LongitudeOfPeriapsis) -> Orbital Elements Bus Creator/9  "Longitude of Periapsis [pi] (rad)"
  Quaternion Conditioner4/1(Qc) -> Quaternions Bus Creator/5, [ICRF2OrbitQ]  "ICRF to Orbit Quaternions"
  MATLAB Function/8(ArgumentOfLatitude) -> Orbital Elements Bus Creator/8  "Argument of Lattitude [u] (rad)"
  Quaternions to Direction Cosine Matrix/1 -> [Orbit2BodyDCM]
  MATLAB Function/1(SemiMajorAxis) -> Orbital Elements Bus Creator/1  "Semi-Major Axis [a] (m)"
  [OrbitalElements] -> ICRF to Body Transfer Matrix Calculator/2(Keplerian Elements)
  Ephemerides [ICRF]1/1 -> Bus Selector3/1
  Dot Product5/1 -> Trigonometric Function1/1
  [ICRF2BodyDCM] -> Transpose/1
  Matrix Multiply2/1 -> Transpose1/1
  Bus Selector1/1 -> MATLAB Function/1(r)  "<Satellite Position [ICRF](m)>"
  ICRF to Body Transfer Matrix Calculator/1(ICRF2BodyTM) -> [ICRF2BodyDCM]
  Orbital Elements Bus Creator/1 -> [OrbitalElements]  "Orbital Elements"
  Transpose1/1 -> [ITRF2BodyDCM]
  Trigonometric Function/1 -> Radians to Degrees4/1
  Constant3/1 -> Dot Product5/2
  [OrbitalElements] -> Transformers Bus Creator/4
  Radians to Degrees4/1 -> Pointing Error Bus Creator/1  "Nadir Pointing Error (deg)"
  Radians to Degrees/1 -> Pointing Error Bus Creator/2  "Sun Pointing Error (deg)"
  Calendar/1 -> ICRF to ITRF DCM Calculator/1(Calendar)  "Calendar"
  Bus Selector4/2 -> Matrix Multiply/2  "<Satellite Position [ICRF](m)>"
  Pointing Error Bus Creator/1 -> [PointingErrors]  "Pinting Error (Deg)"
  [ICRF2BodyQ] -> Virtual Reality World/2(ICRF to Body Quaternions)
  MATLAB Function/11(OrbOmega) -> Orbital Elements Bus Creator/11  "Orbital Frame Angular Velocity {Orbit-ICRF} (rad/s)"
  Constant/1 -> MATLAB Function/3(mu)
  [Orbit2BodyDCM] -> Direction Cosine Matrix to Quaternions2/1  "Orbit to Body TM"
  [ICRF2ITRFDCM] -> TMs Bus Creator/1  "ICRF to ITRF TM"
  [ICRF2BodyDCM] -> TMs Bus Creator/2  "ICRF to Body TM"
  [PointingErrors] -> Transformers Bus Creator/5
  Transpose/1 -> Matrix Multiply2/2
  [Orbit2BodyDCM] -> Product/1
  Direction Cosine Matrix to Quaternions/1 -> Quaternion Conditioner0/1(Q)  "ICRF to Body Quaternions"
  [ICRF2OrbitDCM] -> TMs Bus Creator/5  "ICRF to Orbit TM"
  Quaternion Conditioner/1(Qc) -> Quaternions Bus Creator/6, [ITRF2OrbitQ]  "ITRF to Orbit Quaternions"
  Direction Cosine Matrix to Quaternions3/1 -> Quaternion Conditioner3/1(Q)  "ITRF to Body Quaternions"
  [ICRF2BodyQ] -> Quaternions to Rotation Angles (Euler)2/1
  Constant1/1 -> Product/2, Dot Product1/2
  [ITRF2BodyDCM] -> TMs Bus Creator/4  "ITRF to Body TM"
  Quaternions to Rotation Angles (Euler)7/1 -> Radians to Degrees7/1
  [Quaternions] -> Transformers Bus Creator/2
  [ITRF2OrbitDCM] -> TMs Bus Creator/6  "ITRF to Orbit TM"
  [ICRF2ITRFDCM] -> Matrix Multiply2/1
  Satellite Attitude/1 -> Bus Selector2/1
  Calendar1/1 -> Transformers Bus Creator/6  "Calendar"
  MATLAB Function/2(Eccentricity) -> Orbital Elements Bus Creator/2  "Eccentricity [e]"
  Quaternion Conditioner1/1(Qc) -> Quaternions Bus Creator/2, [ICRF2ITRFQ]  "ICRF to ITRF Quaternions"
  Ephemerides [ICRF]/1 -> Bus Selector1/1
  Quaternions Bus Creator/1 -> [Quaternions]  "Quaternions"
  [ICRF2ITRFDCM] -> Direction Cosine Matrix to Quaternions1/1  "ICRF to ITRF TM"
  Ephemerides [ICRF]2/1 -> Bus Selector4/1
  Direction Cosine Matrix to Quaternions5/1 -> Quaternion Conditioner/1(Q)  "ITRF to Orbit Quaternions"
  Direction Cosine Matrix to Quaternions4/1 -> Quaternion Conditioner4/1(Q)  "ICRF to Orbit Quaternions"
  TMs Bus Creator/1 -> [TransferMatrices]  "Transfer Matrices"
  [ITRF2BodyDCM] -> Direction Cosine Matrix to Quaternions3/1  "ITRF to Body TM"
  Product1/1 -> Dot Product5/1  "Sun Vector [Body] (m)"
  Product/1 -> Dot Product1/1
  Bus Selector2/1 -> Quaternions to Direction Cosine Matrix/1  "<Orbit to Body Quaternions>"
  Quaternion Conditioner3/1(Qc) -> Quaternions Bus Creator/4, [ITRF2BodyQ]  "ITRF to Body Quaternions"
  Direction Cosine Matrix to Quaternions2/1 -> Quaternion Conditioner2/1(Q)  "Orbit to Body Quaternions"
  Quaternion Conditioner0/1(Qc) -> [ICRF2BodyQ], Quaternions Bus Creator/1  "ICRF to Body Quaternions"
  Quaternions to Rotation Angles (Euler)5/1 -> Radians to Degrees5/1
  Dot Product1/1 -> Trigonometric Function/1
  Direction Cosine Matrix to Quaternions1/1 -> Quaternion Conditioner1/1(Q)  "ICRF to ITRF Quaternions"
  Quaternions to Rotation Angles (Euler)2/1 -> Radians to Degrees1/1
  Quaternions to Rotation Angles (Euler)3/1 -> Radians to Degrees2/1
  Euler Angles Bus Creator/1 -> [EulerAngles]  "Euler Angles (deg)"
  MATLAB Function/3(Inclination) -> Orbital Elements Bus Creator/3  "Inclination [i] (rad)"
  [TransferMatrices] -> Transformers Bus Creator/1
  [ICRF2OrbitDCM] -> Direction Cosine Matrix to Quaternions4/1  "ICRF to Orbit TM"
  Quaternions to Rotation Angles (Euler)6/1 -> Radians to Degrees6/1
  [ITRF2BodyQ] -> Quaternions to Rotation Angles (Euler)5/1
  [Orbit2BodyDCM] -> TMs Bus Creator/3  "Orbit to Body TM"
  Trigonometric Function1/1 -> Radians to Degrees/1
  Quaternions to Rotation Angles (Euler)4/1 -> Radians to Degrees3/1
  [ICRF2BodyDCM] -> Direction Cosine Matrix to Quaternions/1  "ICRF to Body TM"
  [Orbit2BodyDCM] -> ICRF to Body Transfer Matrix Calculator/1(Orbit2BodyDCM)
  [ICRF2BodyDCM] -> Product1/1
  Bus Selector3/1 -> Product1/2  "<Sun Position [ICRF] (m)>"
  ICRF to ITRF DCM Calculator/1(ICRF to ITRF DCM) -> [ICRF2ITRFDCM]
  [ICRF2ITRFDCM] -> Matrix Multiply/1  "ICRF to ITRF TM"
  Matrix Multiply/1 -> Virtual Reality World/4(Satellite Position [ITRF] (m))  "Satellite Position [ITRF] (m)"
  [ITRF2BodyQ] -> Virtual Reality World/1(ITRF to Body Quaternions)
  Radians to Degrees1/1 -> Euler Angles Bus Creator/1  "ICRF to Body Euler Angs (deg)"
  Radians to Degrees2/1 -> Euler Angles Bus Creator/2  "ICRF to ITRF Euler Angs (deg)"
  Radians to Degrees3/1 -> Euler Angles Bus Creator/3  "Orbit to Body Euler Angs (deg)"
  Radians to Degrees5/1 -> Euler Angles Bus Creator/4  "ITRF to Body Euler Angs (deg)"
  Radians to Degrees6/1 -> Euler Angles Bus Creator/5  "ICRF to Orbit Euler Angs (deg)"
  Radians to Degrees7/1 -> Euler Angles Bus Creator/6  "ITRF to Orbit Euler Angs (deg)"
  [Orbit2BodyDCM] -> Matrix Multiply3/2
  [ITRF2BodyDCM] -> Transpose4/1
  Matrix Multiply1/1 -> Transpose5/1
  Matrix Multiply3/1 -> Transpose8/1
  [Orbit2BodyDCM] -> Matrix Multiply1/2
  Transpose3/1 -> Matrix Multiply1/1
  [ICRF2BodyDCM] -> Transpose3/1
  Transpose5/1 -> [ICRF2OrbitDCM]
  Transpose8/1 -> [ITRF2OrbitDCM]
  Transpose4/1 -> Matrix Multiply3/1

== system ADCSSimulator/EPS/EPS HouseKeeping/Battery ==
  Battery Capacity (Wh) : Constant  Value=20
  Battery capacity : Outport
  wires:
  Battery Capacity (Wh)/1 -> Battery capacity/1

== system ADCSSimulator/EPS/EPS HouseKeeping/SOC Calculator ==
  Total Current (A) : Inport
  Battery capacity : Inport  Port=2
  Gain : Gain  Gain=3600
  Integrator : Integrator
  MATLAB Function : MATLAB Function  TreatAsAtomicUnit=on
  SOC : Outport
  wires:
  Total Current (A)/1 -> Integrator/1
  Integrator/1 -> MATLAB Function/1(E_used)  "Total Consumed Energy"
  MATLAB Function/1(SOC) -> SOC/1
  Battery capacity/1 -> Gain/1  "W.h"
  Gain/1 -> MATLAB Function/2(E_capacity)  "W.sec"

== system ADCSSimulator/EPS/EPS HouseKeeping/Total Current Consumption (A) ==
  Power Telemetry : Inport
  Bus Selector : BusSelector  OutputSignals=MTQs Power Status.Power Consumption [Magnetorquer X].Current (A),MTQs Power Status.Power Consumption [Magnetorquer Y].Current (A),MTQs Power Status.Power Consumption [Magnetorquer Z].Current (A),RWs Power Status.RW#1 Power Consumption.RW Motor Current (A),RWs Power Status.RW#2 Power Consumption.RW Motor Current (A),RWs Power Status.RW#3 Power Consumption.RW Motor Current (A),RWs Power Status.RW#4 Power Consumption.RW Motor Current (A),Sensors Power Status.Power Consumption [Gyroscope].Current (A),Sensors Power Status.Power Consumption [GNSS Receiver].Current (A),Sensors Power Status.Power Consumption [Magnetometer].Current (A),Sensors Power Status.Power Consumption [Sun Sensor].Current (A)
  Sum : Sum  Inputs=+++++++++++
  Total Current (A) : Outport
  wires:
  Power Telemetry/1 -> Bus Selector/1
  Sum/1 -> Total Current (A)/1
  Bus Selector/1 -> Sum/1  "<Current (A)>"
  Bus Selector/2 -> Sum/2  "<Current (A)>"
  Bus Selector/3 -> Sum/3  "<Current (A)>"
  Bus Selector/4 -> Sum/4  "<RW Motor Current (A)>"
  Bus Selector/5 -> Sum/5  "<RW Motor Current (A)>"
  Bus Selector/6 -> Sum/6  "<RW Motor Current (A)>"
  Bus Selector/7 -> Sum/7  "<RW Motor Current (A)>"
  Bus Selector/8 -> Sum/8  "<Current (A)>"
  Bus Selector/9 -> Sum/9  "<Current (A)>"
  Bus Selector/10 -> Sum/10  "<Current (A)>"
  Bus Selector/11 -> Sum/11  "<Current (A)>"

== system ADCSSimulator/EPS/EPS HouseKeeping/Total Instantaneous Power Consumption (W) ==
  Power Telemetry : Inport
  Bus Selector : BusSelector  OutputSignals=MTQs Power Status.Power Consumption [Magnetorquer X].Power Consumption (W),MTQs Power Status.Power Consumption [Magnetorquer Y].Power Consumption (W),MTQs Power Status.Power Consumption [Magnetorquer Z].Power Consumption (W),RWs Power Status.RW#1 Power Consumption.RW Motor Power Consumption (W),RWs Power Status.RW#2 Power Consumption.RW Motor Power Consumption (W),RWs Power Status.RW#3 Power Consumption.RW Motor Power Consumption (W),RWs Power Status.RW#4 Power Consumption.RW Motor Power Consumption (W),Sensors Power Status.Power Consumption [Gyroscope].Power Consumption (W),Sensors Power Status.Power Consumption [GNSS Receiver].Power Consumption (W),Sensors Power Status.Power Consumption [Magnetometer].Power Consumption (W),Sensors Power Status.Power Consumption [Sun Sensor].Power Consumption (W)
  Sum : Sum  Inputs=+++++++++++
  Total Power Consumption (W) : Outport
  wires:
  Bus Selector/4 -> Sum/4  "<RW Motor Power Consumption (W)>"
  Bus Selector/1 -> Sum/1  "<Power Consumption (W)>"
  Bus Selector/3 -> Sum/3  "<Power Consumption (W)>"
  Bus Selector/10 -> Sum/10  "<Power Consumption (W)>"
  Bus Selector/6 -> Sum/6  "<RW Motor Power Consumption (W)>"
  Bus Selector/9 -> Sum/9  "<Power Consumption (W)>"
  Bus Selector/5 -> Sum/5  "<RW Motor Power Consumption (W)>"
  Bus Selector/11 -> Sum/11  "<Power Consumption (W)>"
  Bus Selector/7 -> Sum/7  "<RW Motor Power Consumption (W)>"
  Bus Selector/2 -> Sum/2  "<Power Consumption (W)>"
  Sum/1 -> Total Power Consumption (W)/1
  Bus Selector/8 -> Sum/8  "<Power Consumption (W)>"
  Power Telemetry/1 -> Bus Selector/1

== system ADCSSimulator/ADCS/ADCS Hardware/Actuators/Reaction Wheels Model (RWs) ==
  RWs Bus Voltage (V) : Inport
  RWs CMD [Body](N.m) : Inport  Port=2
  Angular Velocity Conversion : aerolibconvert2/Angular Velocity Conversion  IU=rad/s  OU=rpm
  Bus Creator : BusCreator  Inputs=3
  Bus Creator3 : BusCreator  Inputs=2
  Reaction Wheel Assembly : Subsystem
  Acutators: RWs : Outport
  wires:
  Reaction Wheel Assembly/1(RWs Torque Out (Nm)) -> Bus Creator/1  "RWs Torque [Body](Nm)"
  Reaction Wheel Assembly/3(RWs Power Status) -> Bus Creator/3  "RWs Power Status"
  RWs CMD [Body](N.m)/1 -> Reaction Wheel Assembly/2(RW Command Torque [Body](N.m))
  RWs Bus Voltage (V)/1 -> Reaction Wheel Assembly/1(RWs Voltage Bus (V))
  Bus Creator/1 -> Acutators: RWs/1
  Bus Creator3/1 -> Bus Creator/2  "RWs Angular Velocity [Body]"
  Angular Velocity Conversion/1 -> Bus Creator3/2  "RWs Angular Velocity (RPM)"
  Reaction Wheel Assembly/2(RWs Angular Velocity (rad/s)) -> Bus Creator3/1, Angular Velocity Conversion/1  "RWs Angular Velocity (rad/s)"
